simulink model "sensor_bias_model"  (R2024b)
settings: Solver=FixedStepDiscrete  StartTime=0.0  StopTime=.2  FixedStep=.001  RelTol=1e-3
model workspace (MAT data in the model file):
  bias_input = timeseries
  bias_input.Name = 'unnamed'
  bias_input.DataInfo = tsdata.datametadata
  bias_input.DataInfo.Interpolation = tsdata.interpolation
  bias_input.DataInfo.Interpolation.Fhandle : function handle (value not decoded)
  bias_input.DataInfo.Interpolation.Name = 'linear'
  bias_input.TimeInfo = tsdata.timemetadata
  bias_input.TimeInfo.Length = 201
  bias_input.TimeInfo.DuplicateTimes = 0
  bias_input.TimeInfo.Time_ = [0; 0.001; 0.002; 0.003; 0.004; 0.005; 0.006; 0.007; 0.008; 0.009; 0.01; 0.011; 0.012; 0.013; 0.014; 0.015; 0.016; 0.017; 0.018; 0.019; 0.02; 0.021; 0.022; 0.023; 0.024; 0.025; 0.026; 0.027; 0.028; 0.029; 0.03; 0.031; 0.032; 0.033; 0.034; 0.035; 0.036; 0.037; 0.038; 0.039; 0.04; 0.041; 0.042; 0.043; 0.044; 0.045; 0.046; 0.047; 0.048; 0.049; 0.05; 0.051; 0.052; 0.053; 0.054; 0.055; 0.056; 0.057; 0.058; 0.059; 0.06; 0.061; 0.062; 0.063; 0.064; 0.065; 0.066; 0.067; 0.068; 0.069; 0.07; 0.071; 0.072; 0.073; 0.074; 0.075; 0.076; 0.077; 0.078; 0.079; 0.08; 0.081; 0.082; 0.083; 0.084; 0.085; 0.086; 0.087; 0.088; 0.089; 0.09; 0.091; 0.092; 0.093; 0.094; 0.095; 0.096; 0.097; 0.098; 0.099; 0.1; 0.101; 0.102; 0.103; 0.104; 0.105; 0.106; 0.107; 0.108; 0.109; 0.11; 0.111; 0.112; 0.113; 0.114; 0.115; 0.116; 0.117; 0.118; 0.119; 0.12; 0.121; 0.122; 0.123; 0.124; 0.125; 0.126; 0.127; 0.128; 0.129; 0.13; 0.131; 0.132; 0.133; 0.134; 0.135; 0.136; 0.137; 0.138; 0.139; 0.14; 0.141; 0.142; 0.143; 0.144; 0.145; 0.146; 0.147; 0.148; 0.149; 0.15; 0.151; 0.152; 0.153; 0.154; 0.155; 0.156; 0.157; 0.158; 0.159; 0.16; 0.161; 0.162; 0.163; 0.164; 0.165; 0.166; 0.167; 0.168; 0.169; 0.17; 0.171; 0.172; 0.173; 0.174; 0.175; 0.176; 0.177; 0.178; 0.179; 0.18; 0.181; 0.182; 0.183; 0.184; 0.185; 0.186; 0.187; 0.188; 0.189; 0.19; 0.191; 0.192; 0.193; 0.194; 0.195; 0.196; 0.197; 0.198; 0.199; 0.2]
  bias_input.TimeInfo.Initialized = 1
  bias_input.QualityInfo = tsdata.qualmetadata
  bias_input.Data_ = [0.004 0.004 0.004 0.004 0.004 0.004 0.004 0.004 0.004 0.004 0.004 0.004 ... (402 elements, 201x2)]
  sensor_input = timeseries
  sensor_input.Name = 'unnamed'
  sensor_input.DataInfo = tsdata.datametadata
  sensor_input.DataInfo.Interpolation = tsdata.interpolation
  sensor_input.DataInfo.Interpolation.Fhandle : function handle (value not decoded)
  sensor_input.DataInfo.Interpolation.Name = 'linear'
  sensor_input.TimeInfo = tsdata.timemetadata
  sensor_input.TimeInfo.Length = 201
  sensor_input.TimeInfo.DuplicateTimes = 0
  sensor_input.TimeInfo.Time_ = [0; 0.001; 0.002; 0.003; 0.004; 0.005; 0.006; 0.007; 0.008; 0.009; 0.01; 0.011; 0.012; 0.013; 0.014; 0.015; 0.016; 0.017; 0.018; 0.019; 0.02; 0.021; 0.022; 0.023; 0.024; 0.025; 0.026; 0.027; 0.028; 0.029; 0.03; 0.031; 0.032; 0.033; 0.034; 0.035; 0.036; 0.037; 0.038; 0.039; 0.04; 0.041; 0.042; 0.043; 0.044; 0.045; 0.046; 0.047; 0.048; 0.049; 0.05; 0.051; 0.052; 0.053; 0.054; 0.055; 0.056; 0.057; 0.058; 0.059; 0.06; 0.061; 0.062; 0.063; 0.064; 0.065; 0.066; 0.067; 0.068; 0.069; 0.07; 0.071; 0.072; 0.073; 0.074; 0.075; 0.076; 0.077; 0.078; 0.079; 0.08; 0.081; 0.082; 0.083; 0.084; 0.085; 0.086; 0.087; 0.088; 0.089; 0.09; 0.091; 0.092; 0.093; 0.094; 0.095; 0.096; 0.097; 0.098; 0.099; 0.1; 0.101; 0.102; 0.103; 0.104; 0.105; 0.106; 0.107; 0.108; 0.109; 0.11; 0.111; 0.112; 0.113; 0.114; 0.115; 0.116; 0.117; 0.118; 0.119; 0.12; 0.121; 0.122; 0.123; 0.124; 0.125; 0.126; 0.127; 0.128; 0.129; 0.13; 0.131; 0.132; 0.133; 0.134; 0.135; 0.136; 0.137; 0.138; 0.139; 0.14; 0.141; 0.142; 0.143; 0.144; 0.145; 0.146; 0.147; 0.148; 0.149; 0.15; 0.151; 0.152; 0.153; 0.154; 0.155; 0.156; 0.157; 0.158; 0.159; 0.16; 0.161; 0.162; 0.163; 0.164; 0.165; 0.166; 0.167; 0.168; 0.169; 0.17; 0.171; 0.172; 0.173; 0.174; 0.175; 0.176; 0.177; 0.178; 0.179; 0.18; 0.181; 0.182; 0.183; 0.184; 0.185; 0.186; 0.187; 0.188; 0.189; 0.19; 0.191; 0.192; 0.193; 0.194; 0.195; 0.196; 0.197; 0.198; 0.199; 0.2]
  sensor_input.TimeInfo.Initialized = 1
  sensor_input.QualityInfo = tsdata.qualmetadata
  sensor_input.Data_ = [0 0.0010048863636 0.00200723429702 0.00300451178242 0.00399419961029 0.0049737977433 0.00594083163154 0.00689285846349 0.00782747333674 0.00874231533302 0.00963507348203 0.0105034925992 ... (402 elements, 201x2)]
settings Model: Creator=Administrator  LastModifiedBy=Administrator

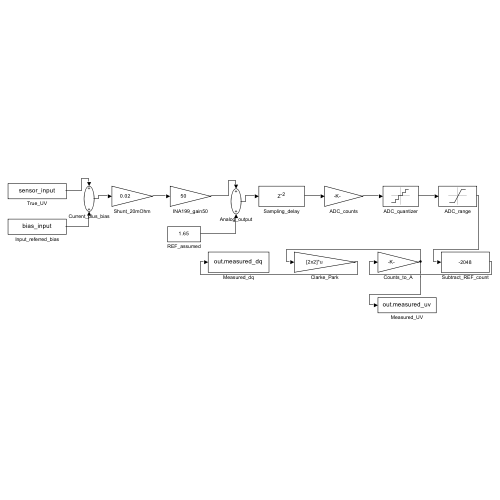
[thumbnail: Simulink's stored preview of the top-level diagram]
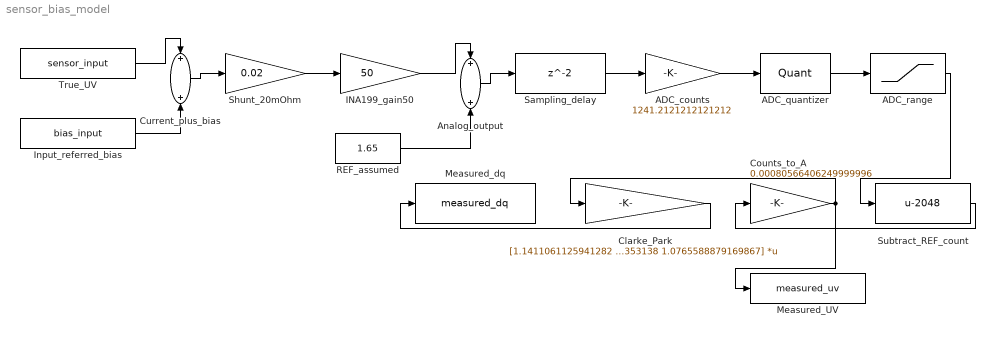
== system sensor_bias_model ==
  ADC_counts : Gain  Gain=1241.2121212121212
  ADC_quantizer : Quantizer  QuantizationInterval=1
  ADC_range : Saturate  UpperLimit=4095  LowerLimit=0
  Analog_output : Sum
  Clarke_Park : Gain  Gain=[1.1411061125941282 0.41755753397618728;0.17666401199353138 1.0765588879169867]  Multiplication=Matrix(K*u)
  Counts_to_A : Gain  Gain=0.00080566406249999996
  Current_plus_bias : Sum
  INA199_gain50 : Gain  Gain=50
  Input_referred_bias : FromWorkspace  VariableName=bias_input
  Measured_UV : ToWorkspace  VariableName=measured_uv  SaveFormat=Timeseries  SampleTime=-1
  Measured_dq : ToWorkspace  VariableName=measured_dq  SaveFormat=Timeseries  SampleTime=-1
  REF_assumed : Constant  Value=1.65
  Sampling_delay : Delay  InitialCondition=[1.6539999999999999 1.6539999999999999;1.6619999999999999 1.6619999999999999]  SampleTime=.001
  Shunt_20mOhm : Gain  Gain=0.02
  Subtract_REF_count : Bias  Bias=-2048  SaturateOnIntegerOverflow=off
  True_UV : FromWorkspace  VariableName=sensor_input
  wires:
  True_UV/1 -> Current_plus_bias/1
  Input_referred_bias/1 -> Current_plus_bias/2
  Current_plus_bias/1 -> Shunt_20mOhm/1
  Shunt_20mOhm/1 -> INA199_gain50/1
  INA199_gain50/1 -> Analog_output/1
  REF_assumed/1 -> Analog_output/2
  Analog_output/1 -> Sampling_delay/1
  Sampling_delay/1 -> ADC_counts/1
  ADC_counts/1 -> ADC_quantizer/1
  ADC_quantizer/1 -> ADC_range/1
  ADC_range/1 -> Subtract_REF_count/1
  Subtract_REF_count/1 -> Counts_to_A/1
  Counts_to_A/1 -> Clarke_Park/1, Measured_UV/1
  Clarke_Park/1 -> Measured_dq/1
